simulink model "FSK"  (R2023b)
settings: Solver=VariableStepAuto  StartTime=0.0  StopTime=30  RelTol=1e-3
libraries: commrandsrc3 x1
settings Model: Creator=lxl  LastModifiedBy=lxl

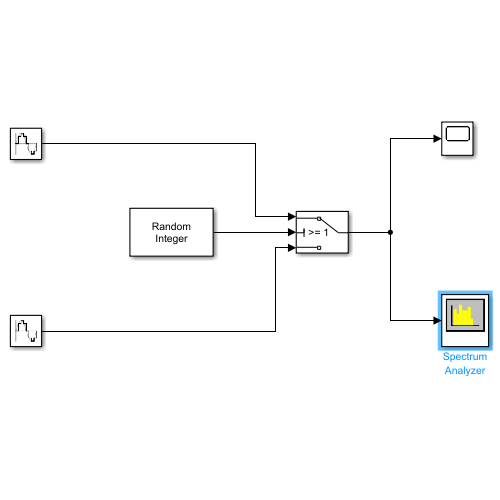
[thumbnail: Simulink's stored preview of the top-level diagram]
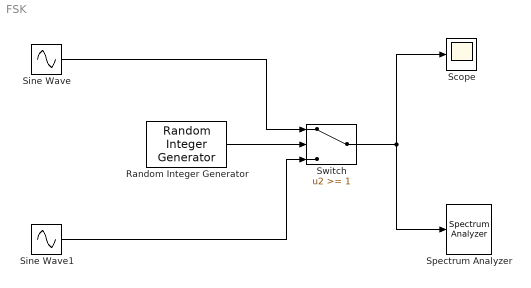
== system FSK ==
  Random Integer Generator : commrandsrc3/Random Integer Generator  SetSize=2  SeedSource=Auto  Seed=0  SampleTime=1  SamplesPerFrame=1  OutputDataType=double  SimulateUsing=Interpreted execution
  Scope : Scope
  Sine Wave : Sin  Frequency=2*pi*10  SampleTime=1/100
  Sine Wave1 : Sin  Frequency=2*pi*5  SampleTime=1/100
  Spectrum Analyzer : SpectrumAnalyzer  WindowPosition=[368.000000,182.000000,800.000000,500.000000,]  Visible=on  ScopeFrameLocation=window
  Switch : Switch  Threshold=1  SaturateOnIntegerOverflow=off  InputSameDT=off
  wires:
  Sine Wave/1 -> Switch/1
  Sine Wave1/1 -> Switch/3
  Random Integer Generator/1 -> Switch/2
  Switch/1 -> Spectrum Analyzer/1, Scope/1
